simulink model "sfVariantLampExample"  (R2025b)
settings: Solver=FixedStepAuto  StartTime=0.0  StopTime=65  RelTol=1e-3
PreLoadFcn:
  | load('sfVariantLampExampleBaseWorkspace.mat')
values from neighbouring files (symbols this model uses):
  HAS_DIMMER1 = 1    [sfVariantLampExampleBaseWorkspace.mat]
  HAS_DIMMER2 = 0    [sfVariantLampExampleBaseWorkspace.mat]
settings Model: Creator=The MathWorks, Inc.  LastModifiedBy=The MathWorks, Inc.
settings SolverCC: AlgebraicLoopSolver=TrustRegion
settings OptimizationCC: DefaultParameterBehavior=Inlined  EnhancedBackFolding=on  PassReuseOutputArgsAs=Individual arguments  ZeroExternalMemoryAtStartup=off  ZeroInternalMemoryAtStartup=off  OptimizeBlockOrder=speed  DifferentSizesBufferReuse=on  OptimizationCustomize=off  EfficientTunableParamExpr=on
settings DebuggingCC: ParameterTunabilityLossMsg=error  UnconnectedInputMsg=warning  UnconnectedOutputMsg=warning  UnconnectedLineMsg=warning
settings ModelReferenceCC: EnableRefExpFcnMdlSchedulingChecks=on
settings SFSimCC: MATLABDynamicMemAlloc=off
settings RTWCC: SystemTargetFile=ert.tlc  TemplateMakefile=ert_default_tmf  GPUComputeCapability=3.5  DLArmComputeVersion=19.05  Description=Embedded Coder
settings CodeAppCC: ForceParamTrailComments=on  IgnoreCustomStorageClasses=off  OperatorAnnotations=on  SimulinkDataObjDesc=on  SFDataObjDesc=on  InsertBlockDesc=on
settings ERTTargetCC: ERTCustomFileTemplate=example_file_process.tlc  DynamicArrayContainerType=coder::array  TargetLangStandard=C99 (ISO)  GenerateSampleERTMain=on

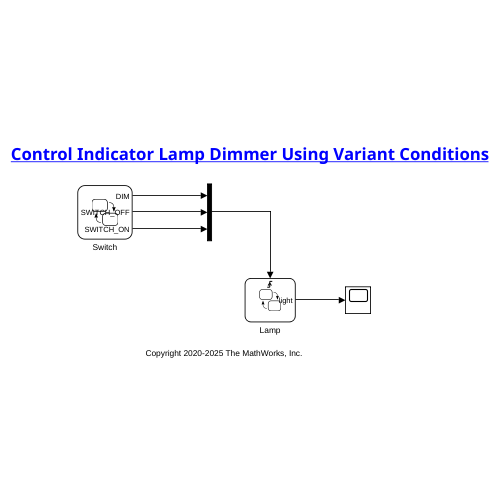
[thumbnail: Simulink's stored preview of the top-level diagram]
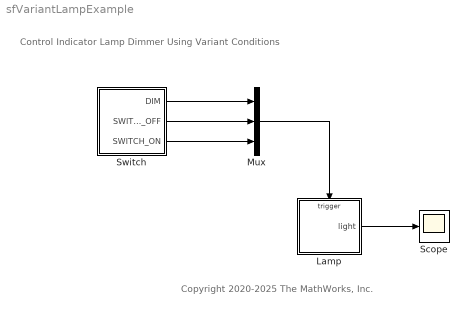
== system sfVariantLampExample ==
  note: Copyright 2020-2025 The MathWorks, Inc.
  note: Control Indicator Lamp Dimmer Using Variant Conditions
  Lamp : Stateflow chart  TreatAsAtomicUnit=on
  Mux : Mux  Inputs=3
  Scope : Scope
      settings: ActiveDisplayYMinimum=-12.5  ActiveDisplayYMaximum=112.5
  Switch : Stateflow chart  TreatAsAtomicUnit=on
  wires:
  Switch/1(DIM) -> Mux/1
  Mux/1 -> Lamp/Trigger
  Lamp/1(light) -> Scope/1
  Switch/2(SWITCH_OFF) -> Mux/2
  Switch/3(SWITCH_ON) -> Mux/3

== stateflow chart sfVariantLampExample/Switch ==
  settings: updateMethod=DISCRETE  sampleTime=1
  state OutsideRoom
  state InsideRoom
    en:
    send(SWITCH_ON)
    du:
    send(DIM)
    exit:
    send(SWITCH_OFF)
  (default) -> OutsideRoom
  InsideRoom -> OutsideRoom : after(50, sec)
  OutsideRoom -> InsideRoom : after(10, sec)
  events: DIM output EITHER_EDGE_EVENT; SWITCH_OFF output EITHER_EDGE_EVENT; SWITCH_ON output EITHER_EDGE_EVENT

== stateflow chart sfVariantLampExample/Lamp ==
  settings: executeAtInitialization=1
  state On
    state Dimmer1
      (history)
      state High
        light = 100;
      state Medium
        light = 75;
      state Low
        light = 25;
      (default) -> On.Dimmer1.High
      On.Dimmer1.High -> Medium : DIM
      Medium -> On.Dimmer1.Low : DIM
      On.Dimmer1.Low -> On.Dimmer1.High : DIM
    state Dimmer2
      (history)
      state High
        light = 100;
      state Low
        light = 50;
      (default) -> On.Dimmer2.High
      On.Dimmer2.High -> On.Dimmer2.Low : DIM
      On.Dimmer2.Low -> On.Dimmer2.High : DIM
    state NoDimmer
      light = 100;
    (default) -> (junction 47)
    (junction 47) -> Dimmer1 [order 1] : [HAS_DIMMER1 == 1]
    (junction 47) -> (junction 50) [order 2]
    (junction 50) -> Dimmer2 [order 1] : [HAS_DIMMER2 == 1]
    (junction 50) -> NoDimmer [order 2]
  state Off
    en:
    light = 0;
  (default) -> Off
  Off -> On : SWITCH_ON
  On -> Off : SWITCH_OFF
  data: light output; HAS_DIMMER1 parameter uint16; HAS_DIMMER2 parameter uint16
  events: DIM input RISING_EDGE_EVENT; SWITCH_OFF input RISING_EDGE_EVENT; SWITCH_ON input RISING_EDGE_EVENT
